simulink model "Model_MapOpt"  (R2023a)
settings: Solver=VariableStepAuto  StartTime=0.0  StopTime=10  MaxStep=0.002  RelTol=1e-6
StopFcn:
  | save_run_results('MapOpt', 'manual_run')
undefined symbols (not defined in the file or in its folder): act_gain_mult, c, C, C_alpha_f, C_col, C_r, ctrl_delay, E, e_c, F_zf, F_zr, Iz, J_col, K, l_f, l_r, m, MapOpt_H_den, MapOpt_H_num, MapOpt_table, MapOpt_Ts_bp, MapOpt_Ts_ctrl, MapOpt_v_bp, motor_wm, n_st, noise_seed_a_y, noise_seed_gamma, noise_seed_T_s, noise_seed_theta1, noise_seed_theta2_dot, noise_seed_v, noise_var_a_y, noise_var_gamma, noise_var_T_s, noise_var_theta1, noise_var_theta2_dot, noise_var_v, sens_Tupd_a_y, sens_Tupd_gamma, sens_Tupd_T_s, sens_Tupd_theta1, sens_Tupd_theta2_dot, sens_Tupd_v, sensors_on, t_0, T_f, Tamax_table, Tamax_v_bp_ms, Tdref_ay_bp_ms2, Tdref_table, Tdref_v_bp_ms
settings Model: Creator=Tan_Tram  LastModifiedBy=Tan_Tram
settings DataIOCC: ReturnWorkspaceOutputs=off

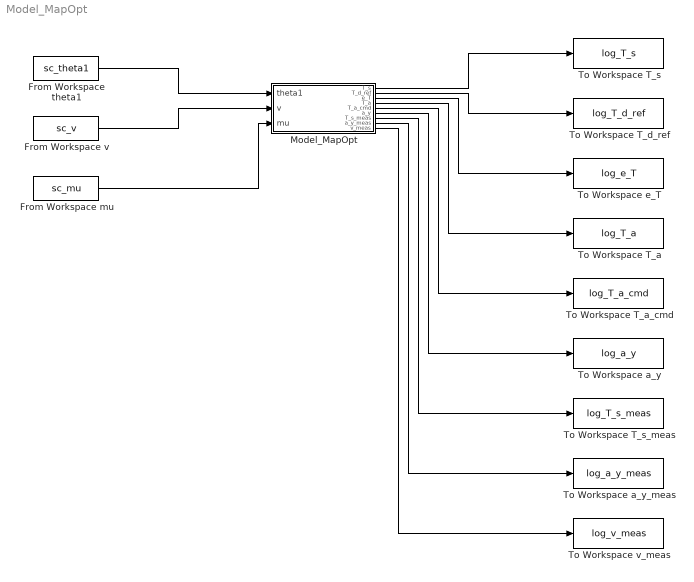
== system Model_MapOpt ==
  From Workspace mu : FromWorkspace  VariableName=sc_mu  OutputAfterFinalValue=Holding final value
  From Workspace theta1 : FromWorkspace  VariableName=sc_theta1  OutputAfterFinalValue=Holding final value
  From Workspace v : FromWorkspace  VariableName=sc_v  OutputAfterFinalValue=Holding final value
  Model_MapOpt : Subsystem
  To Workspace T_a : ToWorkspace  VariableName=log_T_a  SaveFormat=Timeseries  SampleTime=-1
  To Workspace T_a_cmd : ToWorkspace  VariableName=log_T_a_cmd  SaveFormat=Timeseries  SampleTime=-1
  To Workspace T_d_ref : ToWorkspace  VariableName=log_T_d_ref  SaveFormat=Timeseries  SampleTime=-1
  To Workspace T_s : ToWorkspace  VariableName=log_T_s  SaveFormat=Timeseries  SampleTime=-1
  To Workspace T_s_meas : ToWorkspace  VariableName=log_T_s_meas  SaveFormat=Timeseries  SampleTime=-1
  To Workspace a_y : ToWorkspace  VariableName=log_a_y  SaveFormat=Timeseries  SampleTime=-1
  To Workspace a_y_meas : ToWorkspace  VariableName=log_a_y_meas  SaveFormat=Timeseries  SampleTime=-1
  To Workspace e_T : ToWorkspace  VariableName=log_e_T  SaveFormat=Timeseries  SampleTime=-1
  To Workspace v_meas : ToWorkspace  VariableName=log_v_meas  SaveFormat=Timeseries  SampleTime=-1
  wires:
  From Workspace theta1/1 -> Model_MapOpt/1(theta1)
  From Workspace v/1 -> Model_MapOpt/2(v)
  From Workspace mu/1 -> Model_MapOpt/3(mu)
  Model_MapOpt/1(T_s) -> To Workspace T_s/1
  Model_MapOpt/2(T_d_ref) -> To Workspace T_d_ref/1
  Model_MapOpt/3(e_T) -> To Workspace e_T/1
  Model_MapOpt/4(T_a) -> To Workspace T_a/1
  Model_MapOpt/5(T_a_cmd) -> To Workspace T_a_cmd/1
  Model_MapOpt/6(a_y) -> To Workspace a_y/1
  Model_MapOpt/7(T_s_meas) -> To Workspace T_s_meas/1
  Model_MapOpt/8(a_y_meas) -> To Workspace a_y_meas/1
  Model_MapOpt/9(v_meas) -> To Workspace v_meas/1

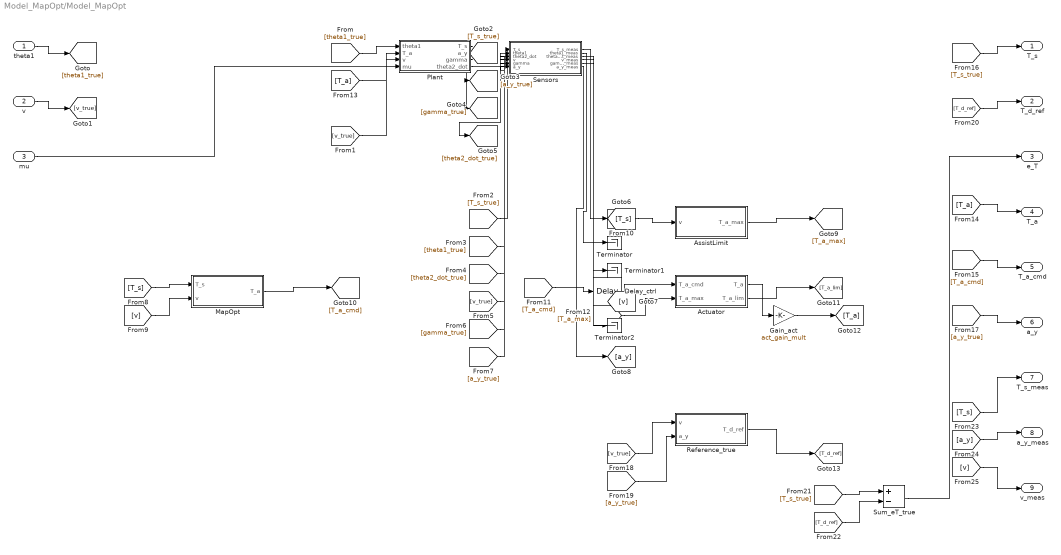
== system Model_MapOpt/Model_MapOpt ==
  theta1 : Inport
  v : Inport  Port=2
  mu : Inport  Port=3
  Actuator : Subsystem
  AssistLimit : Subsystem
  Delay_ctrl : TransportDelay  DelayTime=ctrl_delay
  Gain_act : Gain  Gain=act_gain_mult
  MapOpt : Subsystem
  Plant : Subsystem
  Reference_true : Subsystem
  Sensors : Subsystem
  Sum_eT_true : Sum  Inputs=+-
  Terminator : Terminator
  Terminator1 : Terminator
  Terminator2 : Terminator
  T_s : Outport
  T_d_ref : Outport  Port=2
  e_T : Outport  Port=3
  T_a : Outport  Port=4
  T_a_cmd : Outport  Port=5
  a_y : Outport  Port=6
  T_s_meas : Outport  Port=7
  a_y_meas : Outport  Port=8
  v_meas : Outport  Port=9
  wires:
  theta1/1 -> [theta1_true]
  v/1 -> [v_true]
  mu/1 -> Plant/4(mu)
  [theta1_true] -> Plant/1(theta1)
  [v_true] -> Plant/3(v)
  Plant/1(T_s) -> [T_s_true]
  Plant/2(a_y) -> [a_y_true]
  Plant/3(gamma) -> [gamma_true]
  Plant/4(theta2_dot) -> [theta2_dot_true]
  [T_s_true] -> Sensors/1(T_s)
  [theta1_true] -> Sensors/2(theta1)
  [theta2_dot_true] -> Sensors/3(theta2_dot)
  [v_true] -> Sensors/4(v)
  [gamma_true] -> Sensors/5(gamma)
  [a_y_true] -> Sensors/6(a_y)
  Sensors/1(T_s_meas) -> [T_s]
  Sensors/2(theta1_meas) -> Terminator/1
  Sensors/3(theta2_dot_meas) -> Terminator1/1
  Sensors/4(v_meas) -> [v]
  Sensors/5(gamma_meas) -> Terminator2/1
  Sensors/6(a_y_meas) -> [a_y]
  [T_s] -> MapOpt/1(T_s)
  [v] -> MapOpt/2(v)
  [v] -> AssistLimit/1(v)
  AssistLimit/1(T_a_max) -> [T_a_max]
  MapOpt/1(T_a) -> [T_a_cmd]
  [T_a_cmd] -> Delay_ctrl/1
  Delay_ctrl/1 -> Actuator/1(T_a_cmd)
  [T_a_max] -> Actuator/2(T_a_max)
  Actuator/2(T_a_lim) -> [T_a_lim]
  Actuator/1(T_a) -> Gain_act/1
  Gain_act/1 -> [T_a]
  [T_a] -> Plant/2(T_a)
  [T_a] -> T_a/1
  [T_a_cmd] -> T_a_cmd/1
  [T_s_true] -> T_s/1
  [a_y_true] -> a_y/1
  [v_true] -> Reference_true/1(v)
  [a_y_true] -> Reference_true/2(a_y)
  Reference_true/1(T_d_ref) -> [T_d_ref]
  [T_d_ref] -> T_d_ref/1
  [T_s_true] -> Sum_eT_true/1
  [T_d_ref] -> Sum_eT_true/2
  Sum_eT_true/1 -> e_T/1
  [T_s] -> T_s_meas/1
  [a_y] -> a_y_meas/1
  [v] -> v_meas/1

== system Model_MapOpt/Model_MapOpt/Actuator ==
  T_a_cmd : Inport
  T_a_max : Inport  Port=2
  Cal T_a_lim : Subsystem
  Motor : Subsystem
  T_a : Outport
  T_a_lim : Outport  Port=2
  wires:
  Motor/1(T_a) -> T_a/1
  [T_a_lim] -> Motor/1(T_a_lim)
  [T_a_lim] -> T_a_lim/1
  Cal T_a_lim/1(T_a_lim) -> [T_a_lim]
  [T_a_max] -> Cal T_a_lim/2(T_a_max)
  T_a_cmd/1 -> Cal T_a_lim/1(T_a_cmd)
  T_a_max/1 -> [T_a_max]

== system Model_MapOpt/Model_MapOpt/AssistLimit ==
  v : Inport
  Lookup_Tamax : Lookup_n-D  NumberOfTableDimensions=1  BreakpointsForDimension1=Tamax_v_bp_ms  Table=Tamax_table  ExtrapMethod=Clip  InternalRulePriority=Speed  RndMeth=Simplest
  T_a_max : Outport
  wires:
  Lookup_Tamax/1 -> T_a_max/1
  v/1 -> Lookup_Tamax/1

== system Model_MapOpt/Model_MapOpt/MapOpt ==
  T_s : Inport
  v : Inport  Port=2
  Cal T_a : Subsystem
  Cal T_a_map : Subsystem
  T_a : Outport
  wires:
  Cal T_a/1(T_a) -> T_a/1
  [T_a_map] -> Cal T_a/1(T_a_map)
  Cal T_a_map/1(T_a_map) -> [T_a_map]
  [v] -> Cal T_a_map/2(v)
  v/1 -> [v]
  T_s/1 -> Cal T_a_map/1(T_s)

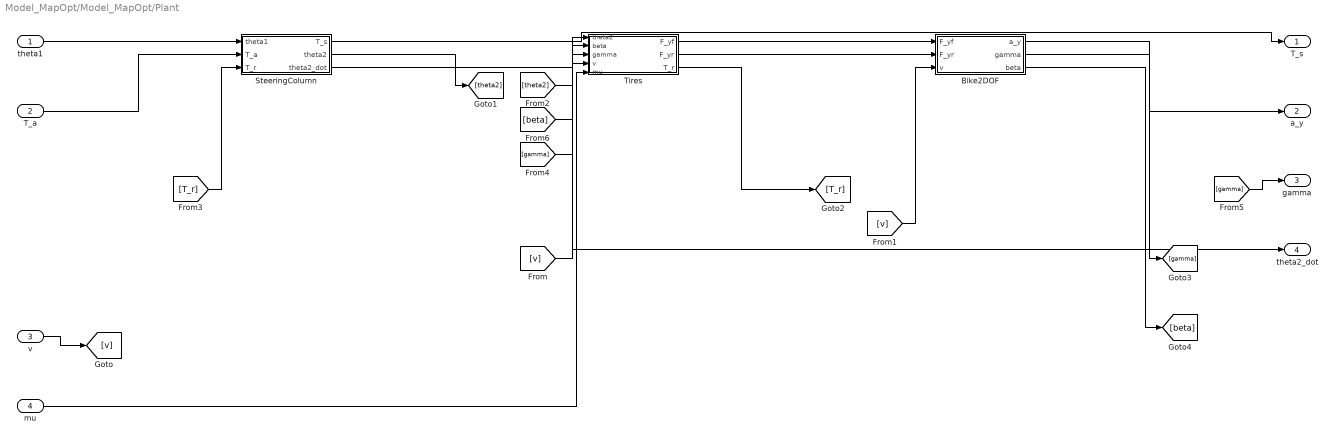
== system Model_MapOpt/Model_MapOpt/Plant ==
  theta1 : Inport
  T_a : Inport  Port=2
  v : Inport  Port=3
  mu : Inport  Port=4
  Bike2DOF : Subsystem
  SteeringColumn : Subsystem
  Tires : Subsystem
  T_s : Outport
  a_y : Outport  Port=2
  gamma : Outport  Port=3
  theta2_dot : Outport  Port=4
  wires:
  [beta] -> Tires/2(beta)
  Bike2DOF/3(beta) -> [beta]
  [gamma] -> gamma/1
  [gamma] -> Tires/3(gamma)
  Bike2DOF/2(gamma) -> [gamma]
  [T_r] -> SteeringColumn/3(T_r)
  Tires/3(T_r) -> [T_r]
  [theta2] -> Tires/1(theta2)
  SteeringColumn/2(theta2) -> [theta2]
  [v] -> Bike2DOF/3(v)
  [v] -> Tires/4(v)
  v/1 -> [v]
  SteeringColumn/3(theta2_dot) -> theta2_dot/1
  Bike2DOF/1(a_y) -> a_y/1
  SteeringColumn/1(T_s) -> T_s/1
  Tires/2(F_yr) -> Bike2DOF/2(F_yr)
  Tires/1(F_yf) -> Bike2DOF/1(F_yf)
  mu/1 -> Tires/5(mu)
  T_a/1 -> SteeringColumn/2(T_a)
  theta1/1 -> SteeringColumn/1(theta1)

== system Model_MapOpt/Model_MapOpt/Reference_true ==
  v : Inport
  a_y : Inport  Port=2
  Cal T_d_ref : Subsystem
  T_d_ref : Outport
  wires:
  Cal T_d_ref/1(T_d_ref) -> T_d_ref/1
  a_y/1 -> Cal T_d_ref/2(a_y)
  v/1 -> Cal T_d_ref/1(v)

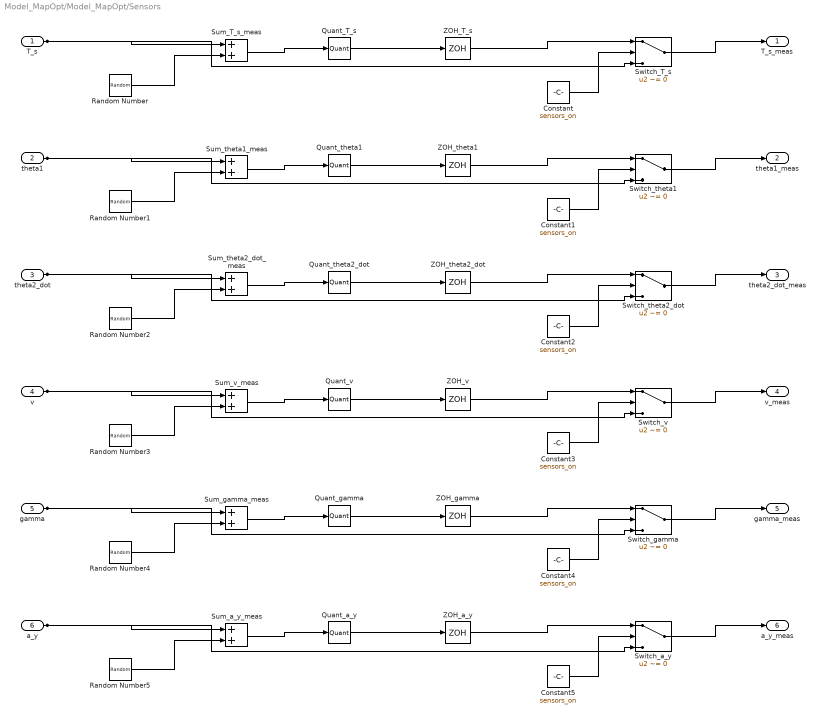
== system Model_MapOpt/Model_MapOpt/Sensors ==
  T_s : Inport
  theta1 : Inport  Port=2
  theta2_dot : Inport  Port=3
  v : Inport  Port=4
  gamma : Inport  Port=5
  a_y : Inport  Port=6
  Constant{,1..5} (6 alike) : Constant  Value=sensors_on
  Quant_T_s : Quantizer  QuantizationInterval=sens_delta_T_s
  Quant_a_y : Quantizer  QuantizationInterval=sens_delta_a_y
  Quant_gamma : Quantizer  QuantizationInterval=sens_delta_gamma
  Quant_theta1 : Quantizer  QuantizationInterval=sens_delta_theta1
  Quant_theta2_dot : Quantizer  QuantizationInterval=sens_delta_theta2_dot
  Quant_v : Quantizer  QuantizationInterval=sens_delta_v
  Random Number : RandomNumber  Variance=noise_var_T_s  Seed=noise_seed_T_s  SampleTime=sens_Tupd_T_s
  Random Number1 : RandomNumber  Variance=noise_var_theta1  Seed=noise_seed_theta1  SampleTime=sens_Tupd_theta1
  Random Number2 : RandomNumber  Variance=noise_var_theta2_dot  Seed=noise_seed_theta2_dot  SampleTime=sens_Tupd_theta2_dot
  Random Number3 : RandomNumber  Variance=noise_var_v  Seed=noise_seed_v  SampleTime=sens_Tupd_v
  Random Number4 : RandomNumber  Variance=noise_var_gamma  Seed=noise_seed_gamma  SampleTime=sens_Tupd_gamma
  Random Number5 : RandomNumber  Variance=noise_var_a_y  Seed=noise_seed_a_y  SampleTime=sens_Tupd_a_y
  Sum_T_s_meas : Sum
  Sum_a_y_meas : Sum
  Sum_gamma_meas : Sum
  Sum_theta1_meas : Sum
  Sum_theta2_dot_meas : Sum
  Sum_v_meas : Sum
  Switch_T_s : Switch  Criteria=u2 ~= 0  SaturateOnIntegerOverflow=off  InputSameDT=off
  Switch_a_y : Switch  Criteria=u2 ~= 0  SaturateOnIntegerOverflow=off  InputSameDT=off
  Switch_gamma : Switch  Criteria=u2 ~= 0  SaturateOnIntegerOverflow=off  InputSameDT=off
  Switch_theta1 : Switch  Criteria=u2 ~= 0  SaturateOnIntegerOverflow=off  InputSameDT=off
  Switch_theta2_dot : Switch  Criteria=u2 ~= 0  SaturateOnIntegerOverflow=off  InputSameDT=off
  Switch_v : Switch  Criteria=u2 ~= 0  SaturateOnIntegerOverflow=off  InputSameDT=off
  ZOH_T_s : ZeroOrderHold  SampleTime=sens_Tupd_T_s
  ZOH_a_y : ZeroOrderHold  SampleTime=sens_Tupd_a_y
  ZOH_gamma : ZeroOrderHold  SampleTime=sens_Tupd_gamma
  ZOH_theta1 : ZeroOrderHold  SampleTime=sens_Tupd_theta1
  ZOH_theta2_dot : ZeroOrderHold  SampleTime=sens_Tupd_theta2_dot
  ZOH_v : ZeroOrderHold  SampleTime=sens_Tupd_v
  T_s_meas : Outport
  theta1_meas : Outport  Port=2
  theta2_dot_meas : Outport  Port=3
  v_meas : Outport  Port=4
  gamma_meas : Outport  Port=5
  a_y_meas : Outport  Port=6
  wires:
  Switch_a_y/1 -> a_y_meas/1
  Constant5/1 -> Switch_a_y/2
  ZOH_a_y/1 -> Switch_a_y/1
  Quant_a_y/1 -> ZOH_a_y/1
  Sum_a_y_meas/1 -> Quant_a_y/1
  Random Number5/1 -> Sum_a_y_meas/2
  a_y/1 -> Switch_a_y/3, Sum_a_y_meas/1
  Switch_gamma/1 -> gamma_meas/1
  Constant4/1 -> Switch_gamma/2
  ZOH_gamma/1 -> Switch_gamma/1
  Quant_gamma/1 -> ZOH_gamma/1
  Sum_gamma_meas/1 -> Quant_gamma/1
  Random Number4/1 -> Sum_gamma_meas/2
  gamma/1 -> Switch_gamma/3, Sum_gamma_meas/1
  Switch_v/1 -> v_meas/1
  Constant3/1 -> Switch_v/2
  ZOH_v/1 -> Switch_v/1
  Quant_v/1 -> ZOH_v/1
  Sum_v_meas/1 -> Quant_v/1
  Random Number3/1 -> Sum_v_meas/2
  v/1 -> Switch_v/3, Sum_v_meas/1
  Switch_theta2_dot/1 -> theta2_dot_meas/1
  Constant2/1 -> Switch_theta2_dot/2
  ZOH_theta2_dot/1 -> Switch_theta2_dot/1
  Quant_theta2_dot/1 -> ZOH_theta2_dot/1
  Sum_theta2_dot_meas/1 -> Quant_theta2_dot/1
  Random Number2/1 -> Sum_theta2_dot_meas/2
  theta2_dot/1 -> Switch_theta2_dot/3, Sum_theta2_dot_meas/1
  Switch_theta1/1 -> theta1_meas/1
  Constant1/1 -> Switch_theta1/2
  ZOH_theta1/1 -> Switch_theta1/1
  Quant_theta1/1 -> ZOH_theta1/1
  Sum_theta1_meas/1 -> Quant_theta1/1
  Random Number1/1 -> Sum_theta1_meas/2
  theta1/1 -> Switch_theta1/3, Sum_theta1_meas/1
  Switch_T_s/1 -> T_s_meas/1
  Constant/1 -> Switch_T_s/2
  ZOH_T_s/1 -> Switch_T_s/1
  Quant_T_s/1 -> ZOH_T_s/1
  Sum_T_s_meas/1 -> Quant_T_s/1
  Random Number/1 -> Sum_T_s_meas/2
  T_s/1 -> Switch_T_s/3, Sum_T_s_meas/1

== system Model_MapOpt/Model_MapOpt/Actuator/Cal T_a_lim ==
  T_a_cmd : Inport
  T_a_max : Inport  Port=2
  Max_Ta : MinMax  Function=max  Inputs=2
  Min_Ta : MinMax  Inputs=2
  Neg_Tamax : UnaryMinus
  T_a_lim : Outport
  wires:
  Max_Ta/1 -> T_a_lim/1
  Neg_Tamax/1 -> Max_Ta/2
  Min_Ta/1 -> Max_Ta/1
  [T_a_max] -> Neg_Tamax/1
  [T_a_max] -> Min_Ta/2
  T_a_cmd/1 -> Min_Ta/1
  T_a_max/1 -> [T_a_max]

== system Model_MapOpt/Model_MapOpt/Actuator/Motor ==
  T_a_lim : Inport
  Motor_lag : TransferFcn  Numerator=[motor_wm]  Denominator=[1 motor_wm]
  T_a : Outport
  wires:
  Motor_lag/1 -> T_a/1
  T_a_lim/1 -> Motor_lag/1

== system Model_MapOpt/Model_MapOpt/MapOpt/Cal T_a ==
  T_a_map : Inport
  Disc_H : DiscreteTransferFcn  Numerator=MapOpt_H_num  Denominator=MapOpt_H_den  SampleTime=MapOpt_Ts_ctrl
  T_a : Outport
  wires:
  Disc_H/1 -> T_a/1
  [T_a_map] -> Disc_H/1
  T_a_map/1 -> [T_a_map]

== system Model_MapOpt/Model_MapOpt/MapOpt/Cal T_a_map ==
  T_s : Inport
  v : Inport  Port=2
  Abs_T_s : Abs  SaturateOnIntegerOverflow=off
  Lookup_M : Lookup_n-D  BreakpointsForDimension1=MapOpt_v_bp  BreakpointsForDimension2=MapOpt_Ts_bp  BreakpointsForDimension3=[5, 7]  Table=MapOpt_table  ExtrapMethod=Clip  InternalRulePriority=Speed  RndMeth=Simplest
      settings: InputPortMap=u0,u1
  Prod_T_a_map : Product  Inputs=**
  Sign_T_s : Signum
  ZOH_T_s : ZeroOrderHold  SampleTime=MapOpt_Ts_ctrl
  ZOH_v : ZeroOrderHold  SampleTime=MapOpt_Ts_ctrl
  T_a_map : Outport
  wires:
  Prod_T_a_map/1 -> T_a_map/1
  Lookup_M/1 -> Prod_T_a_map/2
  Sign_T_s/1 -> Prod_T_a_map/1
  Abs_T_s/1 -> Lookup_M/2
  ZOH_v/1 -> Lookup_M/1
  [T_s] -> Sign_T_s/1
  [T_s] -> Abs_T_s/1
  ZOH_T_s/1 -> [T_s]
  v/1 -> ZOH_v/1
  T_s/1 -> ZOH_T_s/1

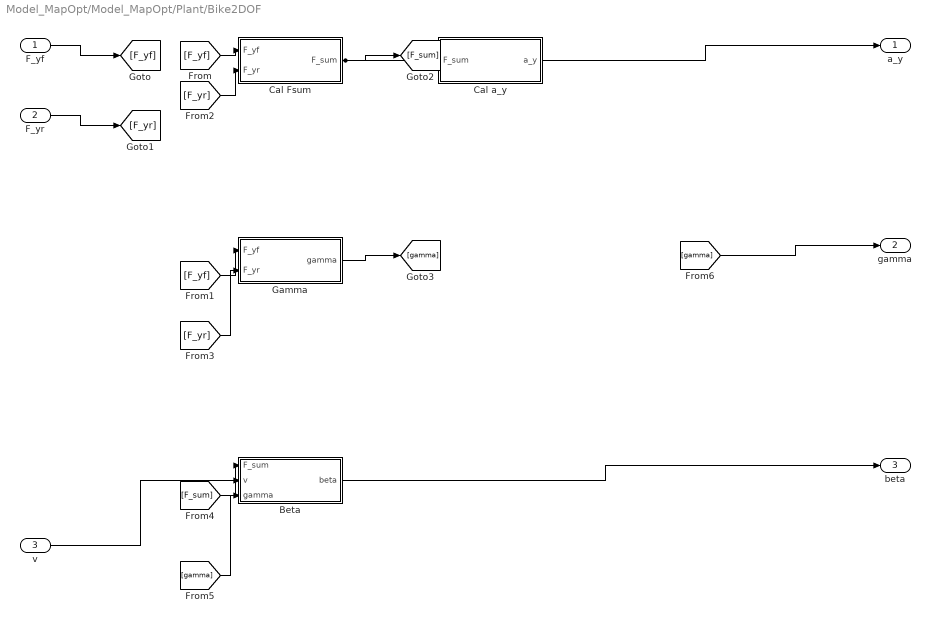
== system Model_MapOpt/Model_MapOpt/Plant/Bike2DOF ==
  F_yf : Inport
  F_yr : Inport  Port=2
  v : Inport  Port=3
  Beta : Subsystem
  Cal Fsum : Subsystem
  Cal a_y : Subsystem
  Gamma : Subsystem
  a_y : Outport
  gamma : Outport  Port=2
  beta : Outport  Port=3
  wires:
  F_yf/1 -> [F_yf]
  [F_yf] -> Cal Fsum/1(F_yf)
  [F_yf] -> Gamma/1(F_yf)
  F_yr/1 -> [F_yr]
  [F_yr] -> Cal Fsum/2(F_yr)
  [F_yr] -> Gamma/2(F_yr)
  Cal Fsum/1(F_sum) -> Cal a_y/1(F_sum), [F_sum]
  [F_sum] -> Beta/1(F_sum)
  Cal a_y/1(a_y) -> a_y/1
  Gamma/1(gamma) -> [gamma]
  [gamma] -> Beta/3(gamma)
  [gamma] -> gamma/1
  v/1 -> Beta/2(v)
  Beta/1(beta) -> beta/1

== system Model_MapOpt/Model_MapOpt/Plant/SteeringColumn ==
  theta1 : Inport
  T_a : Inport  Port=2
  T_r : Inport  Port=3
  Cal T_s : Subsystem
  Lower : Subsystem
  T_s : Outport
  theta2 : Outport  Port=2
  theta2_dot : Outport  Port=3
  wires:
  theta1/1 -> Cal T_s/1(theta1)
  T_a/1 -> Lower/1(T_a)
  T_r/1 -> Lower/2(T_r)
  Lower/2(theta2_dot) -> theta2_dot/1
  Lower/1(theta2) -> [theta2]
  [theta2] -> Cal T_s/2(theta2)
  [theta2] -> theta2/1
  Cal T_s/1(T_s) -> [T_s]
  [T_s] -> Lower/3(T_s)
  [T_s] -> T_s/1

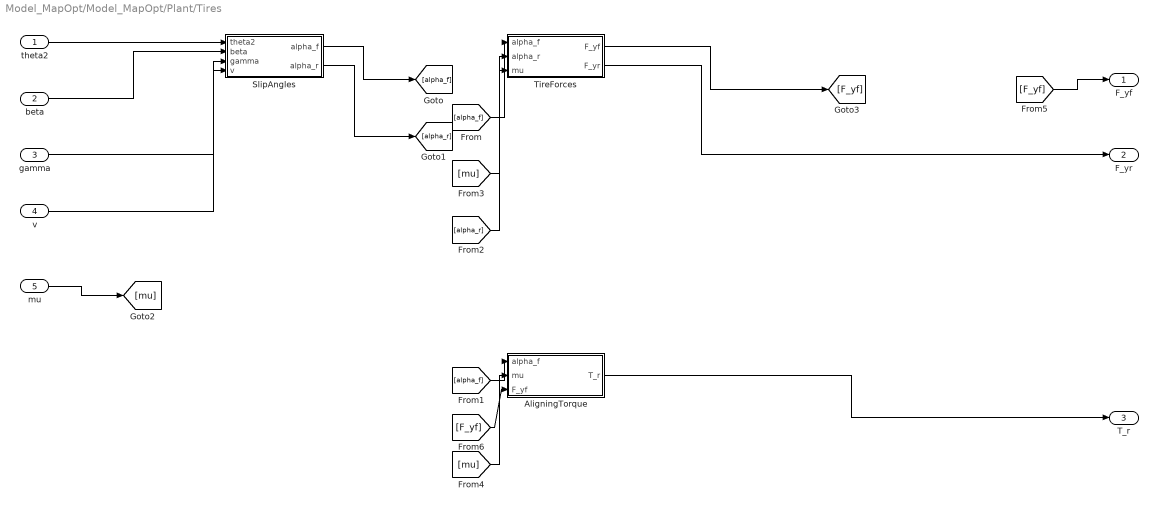
== system Model_MapOpt/Model_MapOpt/Plant/Tires ==
  theta2 : Inport
  beta : Inport  Port=2
  gamma : Inport  Port=3
  v : Inport  Port=4
  mu : Inport  Port=5
  AligningTorque : Subsystem
  SlipAngles : Subsystem
  TireForces : Subsystem
  F_yf : Outport
  F_yr : Outport  Port=2
  T_r : Outport  Port=3
  wires:
  theta2/1 -> SlipAngles/1(theta2)
  beta/1 -> SlipAngles/2(beta)
  gamma/1 -> SlipAngles/3(gamma)
  v/1 -> SlipAngles/4(v)
  SlipAngles/1(alpha_f) -> [alpha_f]
  [alpha_f] -> TireForces/1(alpha_f)
  [alpha_f] -> AligningTorque/1(alpha_f)
  SlipAngles/2(alpha_r) -> [alpha_r]
  [alpha_r] -> TireForces/2(alpha_r)
  mu/1 -> [mu]
  [mu] -> TireForces/3(mu)
  [mu] -> AligningTorque/2(mu)
  TireForces/1(F_yf) -> [F_yf]
  [F_yf] -> F_yf/1
  [F_yf] -> AligningTorque/3(F_yf)
  TireForces/2(F_yr) -> F_yr/1
  AligningTorque/1(T_r) -> T_r/1

== system Model_MapOpt/Model_MapOpt/Reference_true/Cal T_d_ref ==
  v : Inport
  a_y : Inport  Port=2
  Abs_ay : Abs  SaturateOnIntegerOverflow=off
  LUT_Tdref : Lookup_n-D  BreakpointsForDimension1=Tdref_v_bp_ms  BreakpointsForDimension2=Tdref_ay_bp_ms2  Table=Tdref_table  ExtrapMethod=Clip  InternalRulePriority=Speed  RndMeth=Simplest
      settings: InputPortMap=u0,u1
  Prod_Tdref : Product  Inputs=**
  Sign_ay : Signum
  T_d_ref : Outport
  wires:
  Prod_Tdref/1 -> T_d_ref/1
  Sign_ay/1 -> Prod_Tdref/2
  LUT_Tdref/1 -> Prod_Tdref/1
  [a_y] -> Sign_ay/1
  Abs_ay/1 -> LUT_Tdref/2
  [a_y] -> Abs_ay/1
  v/1 -> LUT_Tdref/1
  a_y/1 -> [a_y]

== system Model_MapOpt/Model_MapOpt/Plant/Bike2DOF/Beta ==
  F_sum : Inport
  v : Inport  Port=2
  gamma : Inport  Port=3
  Constant : Constant  Value=m
  Div_Fsum_mv : Product  Inputs=*/
  Int_beta : Integrator
  Prod_mv : Product  Inputs=**
  Sum_betadot : Sum  Inputs=+-
  beta : Outport
  wires:
  Constant/1 -> Prod_mv/1
  v/1 -> Prod_mv/2
  F_sum/1 -> Div_Fsum_mv/1
  Prod_mv/1 -> Div_Fsum_mv/2
  Div_Fsum_mv/1 -> Sum_betadot/1
  gamma/1 -> Sum_betadot/2
  Sum_betadot/1 -> Int_beta/1
  Int_beta/1 -> beta/1

== system Model_MapOpt/Model_MapOpt/Plant/Bike2DOF/Cal Fsum ==
  F_yf : Inport
  F_yr : Inport  Port=2
  Sum_Fsum : Sum
  F_sum : Outport
  wires:
  F_yf/1 -> Sum_Fsum/1
  F_yr/1 -> Sum_Fsum/2
  Sum_Fsum/1 -> F_sum/1

== system Model_MapOpt/Model_MapOpt/Plant/Bike2DOF/Cal a_y ==
  F_sum : Inport
  Constant : Constant  Value=m
  Div_ay : Product  Inputs=*/
  a_y : Outport
  wires:
  F_sum/1 -> Div_ay/1
  Constant/1 -> Div_ay/2
  Div_ay/1 -> a_y/1

== system Model_MapOpt/Model_MapOpt/Plant/Bike2DOF/Gamma ==
  F_yf : Inport
  F_yr : Inport  Port=2
  Constant : Constant  Value=l_f
  Constant1 : Constant  Value=l_r
  Constant2 : Constant  Value=Iz
  Div_gammadot : Product  Inputs=*/
  Int_gamma : Integrator
  Prod_lfFyf : Product  Inputs=**
  Prod_lrFyr : Product  Inputs=**
  Sum_moment : Sum  Inputs=+-
  gamma : Outport
  wires:
  Constant/1 -> Prod_lfFyf/1
  F_yf/1 -> Prod_lfFyf/2
  Constant1/1 -> Prod_lrFyr/1
  F_yr/1 -> Prod_lrFyr/2
  Prod_lfFyf/1 -> Sum_moment/1
  Prod_lrFyr/1 -> Sum_moment/2
  Sum_moment/1 -> Div_gammadot/1
  Constant2/1 -> Div_gammadot/2
  Div_gammadot/1 -> Int_gamma/1
  Int_gamma/1 -> gamma/1

== system Model_MapOpt/Model_MapOpt/Plant/SteeringColumn/Cal T_s ==
  theta1 : Inport
  theta2 : Inport  Port=2
  Constant : Constant  Value=K
  Prod_Ts : Product  Inputs=**
  Sum_dTheta : Sum  Inputs=+-
  T_s : Outport
  wires:
  theta1/1 -> Sum_dTheta/1
  theta2/1 -> Sum_dTheta/2
  Sum_dTheta/1 -> Prod_Ts/1
  Constant/1 -> Prod_Ts/2
  Prod_Ts/1 -> T_s/1

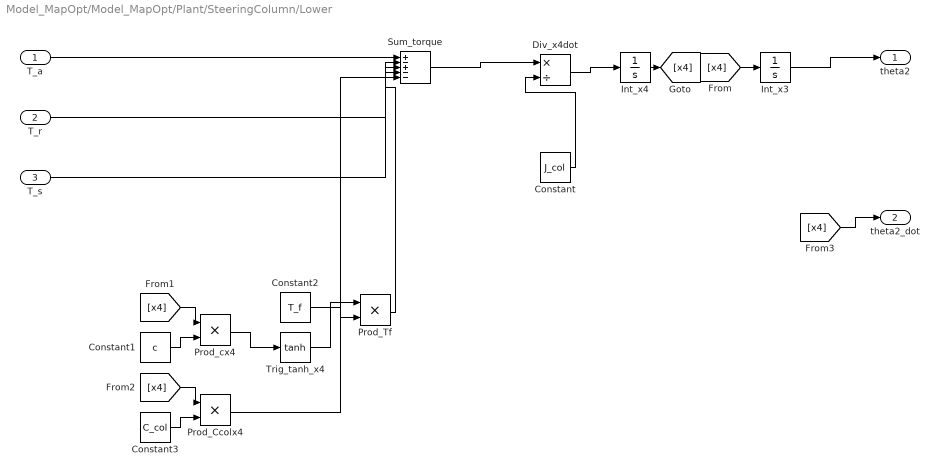
== system Model_MapOpt/Model_MapOpt/Plant/SteeringColumn/Lower ==
  T_a : Inport
  T_r : Inport  Port=2
  T_s : Inport  Port=3
  Constant : Constant  Value=J_col
  Constant1 : Constant  Value=c
  Constant2 : Constant  Value=T_f
  Constant3 : Constant  Value=C_col
  Div_x4dot : Product  Inputs=*/
  Int_x3 : Integrator
  Int_x4 : Integrator
  Prod_Ccolx4 : Product  Inputs=**
  Prod_Tf : Product  Inputs=**
  Prod_cx4 : Product  Inputs=**
  Sum_torque : Sum  Inputs=+-+--
  Trig_tanh_x4 : Trigonometry  Operator=tanh
  theta2 : Outport
  theta2_dot : Outport  Port=2
  wires:
  Int_x4/1 -> [x4]
  [x4] -> Prod_cx4/1
  Constant1/1 -> Prod_cx4/2
  Prod_cx4/1 -> Trig_tanh_x4/1
  Trig_tanh_x4/1 -> Prod_Tf/1
  Constant2/1 -> Prod_Tf/2
  [x4] -> Prod_Ccolx4/1
  Constant3/1 -> Prod_Ccolx4/2
  T_a/1 -> Sum_torque/1
  T_r/1 -> Sum_torque/2
  T_s/1 -> Sum_torque/3
  Prod_Tf/1 -> Sum_torque/4
  Prod_Ccolx4/1 -> Sum_torque/5
  Sum_torque/1 -> Div_x4dot/1
  Constant/1 -> Div_x4dot/2
  Div_x4dot/1 -> Int_x4/1
  [x4] -> Int_x3/1
  Int_x3/1 -> theta2/1
  [x4] -> theta2_dot/1

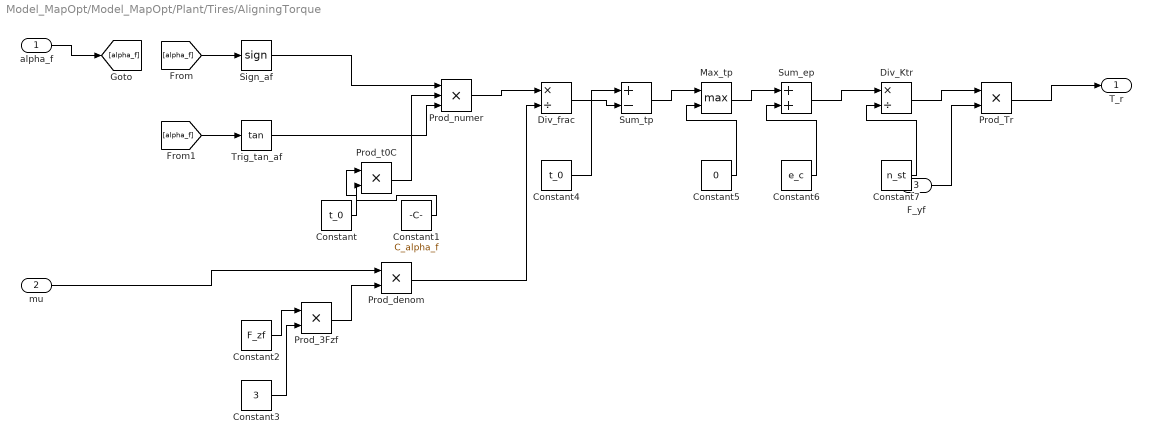
== system Model_MapOpt/Model_MapOpt/Plant/Tires/AligningTorque ==
  alpha_f : Inport
  mu : Inport  Port=2
  F_yf : Inport  Port=3
  Constant : Constant  Value=t_0
  Constant1 : Constant  Value=C_alpha_f
  Constant2 : Constant  Value=F_zf
  Constant3 : Constant  Value=3
  Constant4 : Constant  Value=t_0
  Constant5 : Constant  Value=0
  Constant6 : Constant  Value=e_c
  Constant7 : Constant  Value=n_st
  Div_Ktr : Product  Inputs=*/
  Div_frac : Product  Inputs=*/
  Max_tp : MinMax  Function=max  Inputs=2
  Prod_3Fzf : Product  Inputs=**
  Prod_Tr : Product  Inputs=**
  Prod_denom : Product  Inputs=**
  Prod_numer : Product  Inputs=***
  Prod_t0C : Product  Inputs=**
  Sign_af : Signum
  Sum_ep : Sum
  Sum_tp : Sum  Inputs=+-
  Trig_tan_af : Trigonometry  Operator=tan
  T_r : Outport
  wires:
  alpha_f/1 -> [alpha_f]
  [alpha_f] -> Sign_af/1
  [alpha_f] -> Trig_tan_af/1
  Constant/1 -> Prod_t0C/1
  Constant1/1 -> Prod_t0C/2
  Sign_af/1 -> Prod_numer/1
  Prod_t0C/1 -> Prod_numer/2
  Trig_tan_af/1 -> Prod_numer/3
  Constant2/1 -> Prod_3Fzf/1
  Constant3/1 -> Prod_3Fzf/2
  mu/1 -> Prod_denom/1
  Prod_3Fzf/1 -> Prod_denom/2
  Prod_numer/1 -> Div_frac/1
  Prod_denom/1 -> Div_frac/2
  Constant4/1 -> Sum_tp/1
  Div_frac/1 -> Sum_tp/2
  Sum_tp/1 -> Max_tp/1
  Constant5/1 -> Max_tp/2
  Max_tp/1 -> Sum_ep/1
  Constant6/1 -> Sum_ep/2
  Sum_ep/1 -> Div_Ktr/1
  Constant7/1 -> Div_Ktr/2
  Div_Ktr/1 -> Prod_Tr/1
  F_yf/1 -> Prod_Tr/2
  Prod_Tr/1 -> T_r/1

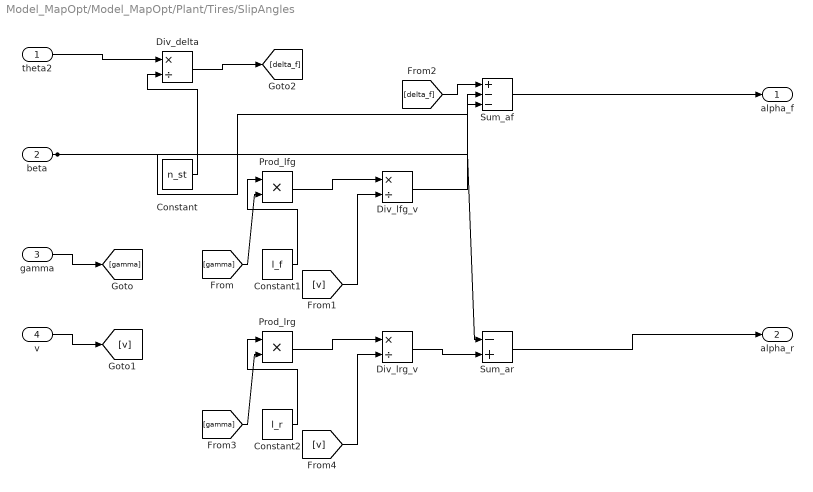
== system Model_MapOpt/Model_MapOpt/Plant/Tires/SlipAngles ==
  theta2 : Inport
  beta : Inport  Port=2
  gamma : Inport  Port=3
  v : Inport  Port=4
  Constant : Constant  Value=n_st
  Constant1 : Constant  Value=l_f
  Constant2 : Constant  Value=l_r
  Div_delta : Product  Inputs=*/
  Div_lfg_v : Product  Inputs=*/
  Div_lrg_v : Product  Inputs=*/
  Prod_lfg : Product  Inputs=**
  Prod_lrg : Product  Inputs=**
  Sum_af : Sum  Inputs=+--
  Sum_ar : Sum  Inputs=-+
  alpha_f : Outport
  alpha_r : Outport  Port=2
  wires:
  gamma/1 -> [gamma]
  v/1 -> [v]
  theta2/1 -> Div_delta/1
  Constant/1 -> Div_delta/2
  Constant1/1 -> Prod_lfg/1
  [gamma] -> Prod_lfg/2
  Prod_lfg/1 -> Div_lfg_v/1
  [v] -> Div_lfg_v/2
  Div_delta/1 -> [delta_f]
  [delta_f] -> Sum_af/1
  beta/1 -> Sum_af/2, Sum_ar/1
  Div_lfg_v/1 -> Sum_af/3
  Sum_af/1 -> alpha_f/1
  Constant2/1 -> Prod_lrg/1
  [gamma] -> Prod_lrg/2
  Prod_lrg/1 -> Div_lrg_v/1
  [v] -> Div_lrg_v/2
  Div_lrg_v/1 -> Sum_ar/2
  Sum_ar/1 -> alpha_r/1

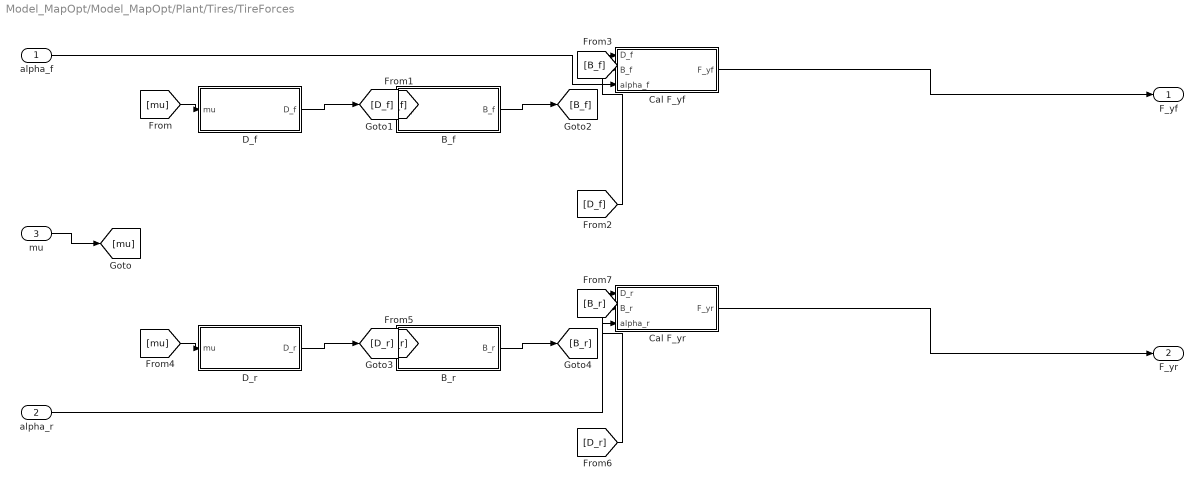
== system Model_MapOpt/Model_MapOpt/Plant/Tires/TireForces ==
  alpha_f : Inport
  alpha_r : Inport  Port=2
  mu : Inport  Port=3
  B_f : Subsystem
  B_r : Subsystem
  Cal F_yf : Subsystem
  Cal F_yr : Subsystem
  D_f : Subsystem
  D_r : Subsystem
  F_yf : Outport
  F_yr : Outport  Port=2
  wires:
  mu/1 -> [mu]
  [mu] -> D_f/1(mu)
  D_f/1(D_f) -> [D_f]
  [D_f] -> B_f/1(D_f)
  [D_f] -> Cal F_yf/1(D_f)
  B_f/1(B_f) -> [B_f]
  [B_f] -> Cal F_yf/2(B_f)
  alpha_f/1 -> Cal F_yf/3(alpha_f)
  Cal F_yf/1(F_yf) -> F_yf/1
  [mu] -> D_r/1(mu)
  D_r/1(D_r) -> [D_r]
  [D_r] -> B_r/1(D_r)
  [D_r] -> Cal F_yr/1(D_r)
  B_r/1(B_r) -> [B_r]
  [B_r] -> Cal F_yr/2(B_r)
  alpha_r/1 -> Cal F_yr/3(alpha_r)
  Cal F_yr/1(F_yr) -> F_yr/1

== system Model_MapOpt/Model_MapOpt/Plant/Tires/TireForces/B_f ==
  D_f : Inport
  Constant : Constant  Value=C
  Constant1 : Constant  Value=C_alpha_f
  Div_B : Product  Inputs=*/
  Prod_CD : Product  Inputs=**
  B_f : Outport
  wires:
  D_f/1 -> Prod_CD/1
  Constant/1 -> Prod_CD/2
  Constant1/1 -> Div_B/1
  Prod_CD/1 -> Div_B/2
  Div_B/1 -> B_f/1

== system Model_MapOpt/Model_MapOpt/Plant/Tires/TireForces/B_r ==
  D_r : Inport
  Constant : Constant  Value=C
  Constant1 : Constant  Value=C_r
  Div_B : Product  Inputs=*/
  Prod_CD : Product  Inputs=**
  B_r : Outport
  wires:
  D_r/1 -> Prod_CD/1
  Constant/1 -> Prod_CD/2
  Constant1/1 -> Div_B/1
  Prod_CD/1 -> Div_B/2
  Div_B/1 -> B_r/1

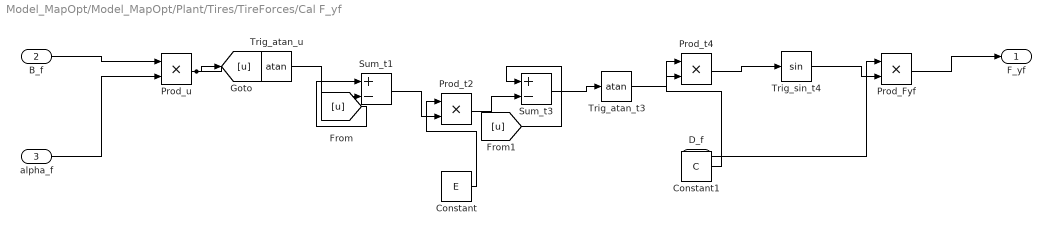
== system Model_MapOpt/Model_MapOpt/Plant/Tires/TireForces/Cal F_yf ==
  D_f : Inport
  B_f : Inport  Port=2
  alpha_f : Inport  Port=3
  Constant : Constant  Value=E
  Constant1 : Constant  Value=C
  Prod_Fyf : Product  Inputs=**
  Prod_t2 : Product  Inputs=**
  Prod_t4 : Product  Inputs=**
  Prod_u : Product  Inputs=**
  Sum_t1 : Sum  Inputs=+-
  Sum_t3 : Sum  Inputs=+-
  Trig_atan_t3 : Trigonometry  Operator=atan
  Trig_atan_u : Trigonometry  Operator=atan
  Trig_sin_t4 : Trigonometry
  F_yf : Outport
  wires:
  B_f/1 -> Prod_u/1
  alpha_f/1 -> Prod_u/2
  Prod_u/1 -> Trig_atan_u/1, [u]
  [u] -> Sum_t1/1
  Trig_atan_u/1 -> Sum_t1/2
  Constant/1 -> Prod_t2/1
  Sum_t1/1 -> Prod_t2/2
  [u] -> Sum_t3/1
  Prod_t2/1 -> Sum_t3/2
  Sum_t3/1 -> Trig_atan_t3/1
  Constant1/1 -> Prod_t4/1
  Trig_atan_t3/1 -> Prod_t4/2
  Prod_t4/1 -> Trig_sin_t4/1
  D_f/1 -> Prod_Fyf/1
  Trig_sin_t4/1 -> Prod_Fyf/2
  Prod_Fyf/1 -> F_yf/1

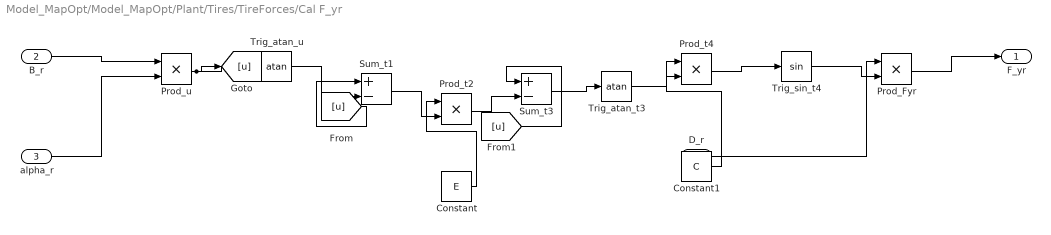
== system Model_MapOpt/Model_MapOpt/Plant/Tires/TireForces/Cal F_yr ==
  D_r : Inport
  B_r : Inport  Port=2
  alpha_r : Inport  Port=3
  Constant : Constant  Value=E
  Constant1 : Constant  Value=C
  Prod_Fyr : Product  Inputs=**
  Prod_t2 : Product  Inputs=**
  Prod_t4 : Product  Inputs=**
  Prod_u : Product  Inputs=**
  Sum_t1 : Sum  Inputs=+-
  Sum_t3 : Sum  Inputs=+-
  Trig_atan_t3 : Trigonometry  Operator=atan
  Trig_atan_u : Trigonometry  Operator=atan
  Trig_sin_t4 : Trigonometry
  F_yr : Outport
  wires:
  B_r/1 -> Prod_u/1
  alpha_r/1 -> Prod_u/2
  Prod_u/1 -> Trig_atan_u/1, [u]
  [u] -> Sum_t1/1
  Trig_atan_u/1 -> Sum_t1/2
  Constant/1 -> Prod_t2/1
  Sum_t1/1 -> Prod_t2/2
  [u] -> Sum_t3/1
  Prod_t2/1 -> Sum_t3/2
  Sum_t3/1 -> Trig_atan_t3/1
  Constant1/1 -> Prod_t4/1
  Trig_atan_t3/1 -> Prod_t4/2
  Prod_t4/1 -> Trig_sin_t4/1
  D_r/1 -> Prod_Fyr/1
  Trig_sin_t4/1 -> Prod_Fyr/2
  Prod_Fyr/1 -> F_yr/1

== system Model_MapOpt/Model_MapOpt/Plant/Tires/TireForces/D_f ==
  mu : Inport
  Constant : Constant  Value=F_zf
  Prod_D : Product  Inputs=**
  D_f : Outport
  wires:
  mu/1 -> Prod_D/1
  Constant/1 -> Prod_D/2
  Prod_D/1 -> D_f/1

== system Model_MapOpt/Model_MapOpt/Plant/Tires/TireForces/D_r ==
  mu : Inport
  Constant : Constant  Value=F_zr
  Prod_D : Product  Inputs=**
  D_r : Outport
  wires:
  mu/1 -> Prod_D/1
  Constant/1 -> Prod_D/2
  Prod_D/1 -> D_r/1
